simulink model "sfHierarchyAPIExample"  (R2025b)
settings: Solver=VariableStepAuto  StartTime=0.0  StopTime=10.0  RelTol=1e-3
settings Model: Creator=The MathWorks, Inc.  LastModifiedBy=The MathWorks, Inc.
settings OptimizationCC: ReuseModelBlockBuffer=off
settings RTWCC: GPUComputeCapability=3.5

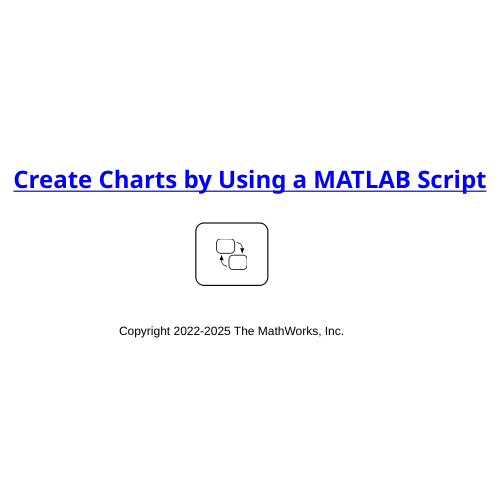
[thumbnail: Simulink's stored preview of the top-level diagram]
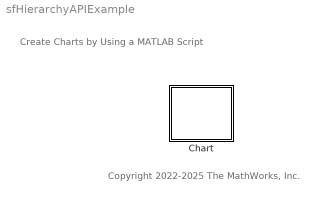
== system sfHierarchyAPIExample ==
  note: Copyright 2022-2025 The MathWorks, Inc.
  note: Create Charts by Using a MATLAB Script
  Chart : Stateflow chart  TreatAsAtomicUnit=on

== stateflow chart sfHierarchyAPIExample/Chart ==
  state A
    state A1
    state A2
    (default) -> A1
    A1 -> A2
  (default) -> A
